simulink model "OFWTmodel"  (R2020a)
settings: Solver=ode4  StartTime=0  StopTime=800  FixedStep=0.05  MaxStep=0.05  RelTol=1e-3
undefined symbols (not defined in the file or in its folder): body, constraint, geometry, hydroData, mooring, windTurbine
libraries: WECSim_Lib_Constraints x1, WECSim_Lib_Frames x1, WECSim_Lib_Moorings x1, WECSim_Lib_Body_Elements x1, MOST_Lib x1
settings Model: Creator=massi  LastModifiedBy=emili
settings SolverCC: ZeroCrossControl=DisableAll  AutoInsertRateTranBlk=on
settings DataIOCC: ReturnWorkspaceOutputs=off
settings OptimizationCC: SimCompilerOptimization=on
settings ExplorerConfigSet: SimMechanicsOpenEditorOnUpdate=off  InternalSimMechanicsExplorerSettings="<ExplorerConfiguration><canonicalview>default</canonicalview><AnimationSetting><BasePlaybackSpeed>1.0</BasePlaybackSpeed><PlaybackSpeedFactor>64.0</PlaybackSpeedFactor></AnimationSetting><TilePanel><TileInfo><Tiles Columns=\"1\" Count=\"1\" Rows=\"1\"><Column Weight=\"1\"/><Row Weight=\"1\"/><Tile Height=\"1\" Width=\"1\" X=\"0\" Y=\"0\"/></Tiles></TileInfo><SceneInfo><SceneViewer><BGColor><R>0.800000011920928955</R><G>1</G><B>1</B></BGColor><Camera><DoPerspective>off</DoPerspective><Position><X>3.83527572012098972e-06</X><Y>-435.132249170182718</Y><Z>-23.2456610583153065</Z></Position><Center><X>3.83527572012098972e-06</X><Y>-1.30964724540660882e-05</Y><Z>-23.2456610583153065</Z></Center><Up><X>0</X><Y>-0</Y><Z>1</Z></Up><ViewLimDist>1</ViewLimDist><YLim>286.086963500976594</YLim><XLim>444.426516742997762</XLim></Camera></SceneViewer></SceneInfo></TilePanel><MechEditorPanel><Cameras/><GfxPanelCameraMap/><VideoCreator><PlaybackSpeedRatio>1.0</PlaybackSpeedRatio><FrameRate>30</FrameRate><VideoFormat>Motion JPEG AVI</VideoFormat><FrameSize>auto</FrameSize></VideoCreator></MechEditorPanel></ExplorerConfiguration>"

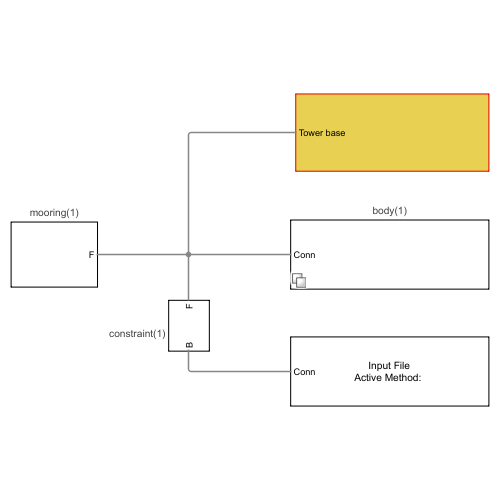
[thumbnail: Simulink's stored preview of the top-level diagram]
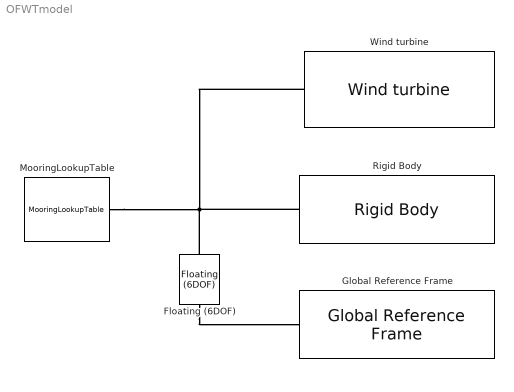
== system OFWTmodel ==
  Floating (6DOF) : WECSim_Lib_Constraints/Floating (6DOF)  constraint=constraint(1)  loc="0  0  0"  displacement=0 0 0  y=0 1 0  z=0 0 1  upperLimitSpecify=off  upperLimitBound=0  upperLimitTransitionRegionWidth=0  upperLimitStiffness=0  upperLimitDamping=0  lowerLimitSpecify=off  lowerLimitBound=0  lowerLimitTransitionRegionWidth=0  lowerLimitStiffness=0  lowerLimitDamping=0
      settings: AttributesFormatString=%<constraint>
  Global Reference Frame : WECSim_Lib_Frames/Global Reference Frame  waves=waves  simu=simu  InputMethod=Input File  InputFile=wecSimInputFile.m  mode=normal  explorer=off  solver=ode4  startTime=0  rampTime=100  endTime=400  dt=0.1  cicEndTime=60  stateSpace=0  WaveClass=regular  height=2.5  period=8  elevationFile=NOT DEFINED  spectrumFile=NOT DEFINED  direction=0  spread=1  spectrumType=NOT DEFINED  phaseSeed=0  option=EqualEnergy
  MooringLookupTable : WECSim_Lib_Moorings/MooringLookupTable  mooring=mooring(1)
      settings: AttributesFormatString=%<mooring>
  Rigid Body : WECSim_Lib_Body_Elements/Rigid Body  body=body(1)  h5File=hydroData/*.h5  geometryFile=geometry/*.stl  mass=0  inertia=0 0 0  inertiaProducts=0 0 0  nonHydro=0  nonlinearHydro=0  centerGravity=0 0 0  centerBuoyancy=0 0 0  dof=6  volume=0  displacement=0 0 0  axis=0 1 0  angle=0  option=0  cd=0 0 0  ca=0 0 0  area=0 0 0  VME=0  rgME=0 0 0  z=0 0 1
  Wind turbine : MOST_Lib/Wind turbine  VariantControl=sv_1_IEA15MW  windTurbine=windTurbine(1)
      settings: SourceProductName=MOST
  connections:
  Floating (6DOF)/LConn1 -- Global Reference Frame/RConn1
  Rigid Body/RConn1 -- Floating (6DOF)/RConn1 -- MooringLookupTable/LConn1 -- Wind turbine/RConn1
